simulink model "QuadArchitecture_AI"  (R2026b)
settings: Solver=VariableStepAuto
settings Model: DataDictionary=QuadInterfaces_AI.sldd  Creator=JonathanTee  LastModifiedBy=JonathanTee

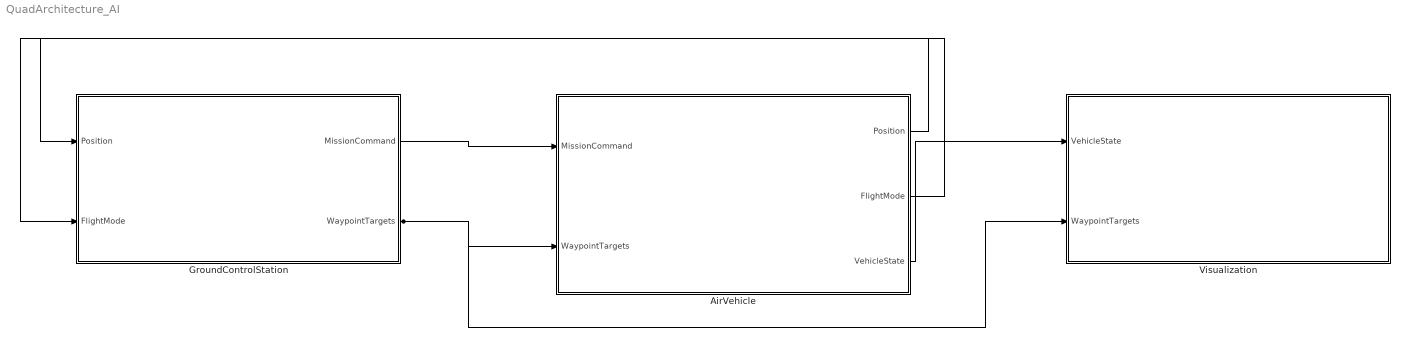
== system QuadArchitecture_AI ==
  AirVehicle : Subsystem
      settings: PortSchema="{\"entries\":[{\"content\":{\"headerSize\":26,\"margin\":15,\"minimumSpacing\":25,\"sides\":[{\"content\":{\"connectorIds\":[\"In1\",\"In2\"]},\"type\":\"ConnectorPlacement.EquallySpacedRectSide\",\"uuid\":\"ecfb2a5d-ebc3-4605-9a84-c6fd342510eb\"},{\"content\":{\"connectorIds\":[\"Out1\",\"Out2\",\"Out3\"],\"side\":\"RIGHT\"},\"type\":\"ConnectorPlacement.EquallySpacedRectSide\",\"uuid\":\"41ea779c-ccae-40c9-bf4c-62eb2a12d4ec\"},{\"content\":{\"side\":\"TOP\"},\"type\":\"ConnectorPlacement.EquallySpacedRectSide\",\"uuid\":\"f1fc56fa-babc-4d23-97d2-f02afcdd55d8\"}]},\"type\":\"ConnectorPlacement.EquallySpacedConnector\",\"uuid\":\"2007e49f-3d37-456e-85ff-e7f0d83353ae\"}],\"packageUris\":[\"http://schema.mathworks.com/mf0/Connector/R2020b\"],\"version\":\"1.0\"}"
  GroundControlStation : Subsystem
      settings: PortSchema="{\"entries\":[{\"content\":{\"headerSize\":26,\"margin\":15,\"minimumSpacing\":25,\"sides\":[{\"content\":{\"connectorIds\":[\"In1\",\"In2\"]},\"type\":\"ConnectorPlacement.EquallySpacedRectSide\",\"uuid\":\"ecfb2a5d-ebc3-4605-9a84-c6fd342510eb\"},{\"content\":{\"connectorIds\":[\"Out1\",\"Out2\"],\"side\":\"RIGHT\"},\"type\":\"ConnectorPlacement.EquallySpacedRectSide\",\"uuid\":\"41ea779c-ccae-40c9-bf4c-62eb2a12d4ec\"},{\"content\":{\"side\":\"TOP\"},\"type\":\"ConnectorPlacement.EquallySpacedRectSide\",\"uuid\":\"f1fc56fa-babc-4d23-97d2-f02afcdd55d8\"}]},\"type\":\"ConnectorPlacement.EquallySpacedConnector\",\"uuid\":\"2007e49f-3d37-456e-85ff-e7f0d83353ae\"}],\"packageUris\":[\"http://schema.mathworks.com/mf0/Connector/R2020b\"],\"version\":\"1.0\"}"
  Visualization : Subsystem
      settings: PortSchema="{\"entries\":[{\"content\":{\"headerSize\":26,\"margin\":15,\"minimumSpacing\":25,\"sides\":[{\"content\":{\"connectorIds\":[\"In1\",\"In2\"]},\"type\":\"ConnectorPlacement.EquallySpacedRectSide\",\"uuid\":\"ecfb2a5d-ebc3-4605-9a84-c6fd342510eb\"},{\"content\":{\"side\":\"RIGHT\"},\"type\":\"ConnectorPlacement.EquallySpacedRectSide\",\"uuid\":\"41ea779c-ccae-40c9-bf4c-62eb2a12d4ec\"},{\"content\":{\"side\":\"TOP\"},\"type\":\"ConnectorPlacement.EquallySpacedRectSide\",\"uuid\":\"f1fc56fa-babc-4d23-97d2-f02afcdd55d8\"}]},\"type\":\"ConnectorPlacement.EquallySpacedConnector\",\"uuid\":\"2007e49f-3d37-456e-85ff-e7f0d83353ae\"}],\"packageUris\":[\"http://schema.mathworks.com/mf0/Connector/R2020b\"],\"version\":\"1.0\"}"
  wires:
  AirVehicle/3(VehicleState) -> Visualization/1(VehicleState)
  AirVehicle/2(FlightMode) -> GroundControlStation/2(FlightMode)
  AirVehicle/1(Position) -> GroundControlStation/1(Position)
  GroundControlStation/2(WaypointTargets) -> Visualization/2(WaypointTargets), AirVehicle/2(WaypointTargets)
  GroundControlStation/1(MissionCommand) -> AirVehicle/1(MissionCommand)

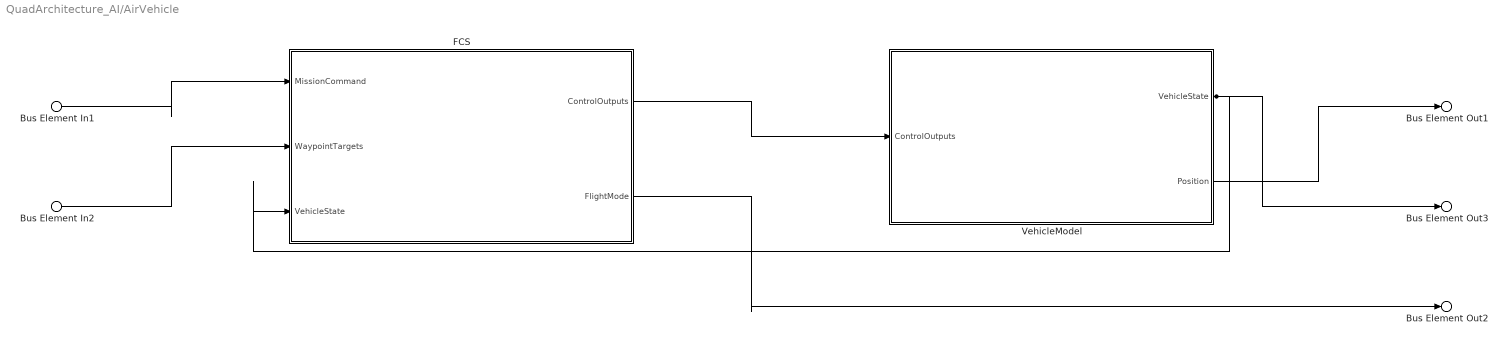
== system QuadArchitecture_AI/AirVehicle ==
  Bus Element In1 : Inport  PortName=MissionCommand
  Bus Element In2 : Inport  Port=2  PortName=WaypointTargets
  FCS : Subsystem
      settings: PortSchema="{\"entries\":[{\"content\":{\"headerSize\":26,\"margin\":15,\"minimumSpacing\":25,\"sides\":[{\"content\":{\"connectorIds\":[\"In1\",\"In2\",\"In3\"]},\"type\":\"ConnectorPlacement.EquallySpacedRectSide\",\"uuid\":\"ecfb2a5d-ebc3-4605-9a84-c6fd342510eb\"},{\"content\":{\"connectorIds\":[\"Out1\",\"Out2\"],\"side\":\"RIGHT\"},\"type\":\"ConnectorPlacement.EquallySpacedRectSide\",\"uuid\":\"41ea779c-ccae-40c9-bf4c-62eb2a12d4ec\"},{\"content\":{\"side\":\"TOP\"},\"type\":\"ConnectorPlacement.EquallySpacedRectSide\",\"uuid\":\"f1fc56fa-babc-4d23-97d2-f02afcdd55d8\"}]},\"type\":\"ConnectorPlacement.EquallySpacedConnector\",\"uuid\":\"2007e49f-3d37-456e-85ff-e7f0d83353ae\"}],\"packageUris\":[\"http://schema.mathworks.com/mf0/Connector/R2020b\"],\"version\":\"1.0\"}"
  VehicleModel : Subsystem
      settings: PortSchema="{\"entries\":[{\"content\":{\"headerSize\":26,\"margin\":15,\"minimumSpacing\":25,\"sides\":[{\"content\":{\"connectorIds\":[\"In1\"]},\"type\":\"ConnectorPlacement.EquallySpacedRectSide\",\"uuid\":\"ecfb2a5d-ebc3-4605-9a84-c6fd342510eb\"},{\"content\":{\"connectorIds\":[\"Out1\",\"Out2\"],\"side\":\"RIGHT\"},\"type\":\"ConnectorPlacement.EquallySpacedRectSide\",\"uuid\":\"41ea779c-ccae-40c9-bf4c-62eb2a12d4ec\"},{\"content\":{\"side\":\"TOP\"},\"type\":\"ConnectorPlacement.EquallySpacedRectSide\",\"uuid\":\"f1fc56fa-babc-4d23-97d2-f02afcdd55d8\"}]},\"type\":\"ConnectorPlacement.EquallySpacedConnector\",\"uuid\":\"2007e49f-3d37-456e-85ff-e7f0d83353ae\"}],\"packageUris\":[\"http://schema.mathworks.com/mf0/Connector/R2020b\"],\"version\":\"1.0\"}"
  Bus Element Out1 : Outport  PortName=Position
  Bus Element Out2 : Outport  Port=2  PortName=FlightMode
  Bus Element Out3 : Outport  Port=3  PortName=VehicleState
  wires:
  FCS/2(FlightMode) -> Bus Element Out2/1
  VehicleModel/2(Position) -> Bus Element Out1/1
  VehicleModel/1(VehicleState) -> Bus Element Out3/1, FCS/3(VehicleState)
  FCS/1(ControlOutputs) -> VehicleModel/1(ControlOutputs)
  Bus Element In2/1 -> FCS/2(WaypointTargets)
  Bus Element In1/1 -> FCS/1(MissionCommand)

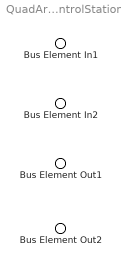
== system QuadArchitecture_AI/GroundControlStation ==
  Bus Element In1 : Inport  PortName=Position
  Bus Element In2 : Inport  Port=2  PortName=FlightMode
  Bus Element Out1 : Outport  PortName=MissionCommand
  Bus Element Out2 : Outport  Port=2  PortName=WaypointTargets

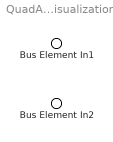
== system QuadArchitecture_AI/Visualization ==
  Bus Element In1 : Inport  PortName=VehicleState
  Bus Element In2 : Inport  Port=2  PortName=WaypointTargets

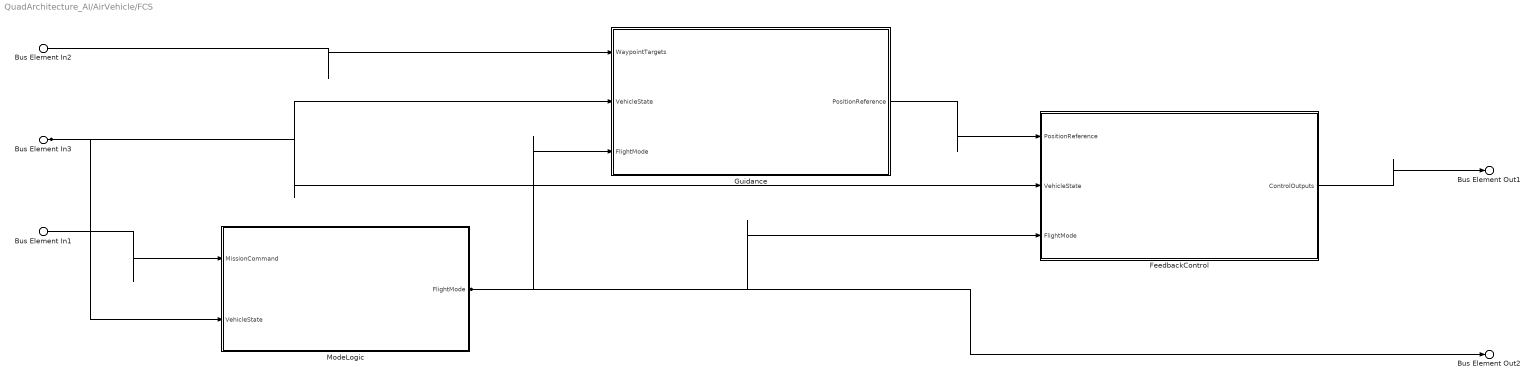
== system QuadArchitecture_AI/AirVehicle/FCS ==
  Bus Element In1 : Inport  PortName=MissionCommand
  Bus Element In2 : Inport  Port=2  PortName=WaypointTargets
  Bus Element In3 : Inport  Port=3  PortName=VehicleState
  FeedbackControl : Subsystem
      settings: PortSchema="{\"entries\":[{\"content\":{\"headerSize\":26,\"margin\":15,\"minimumSpacing\":25,\"sides\":[{\"content\":{\"connectorIds\":[\"In1\",\"In2\",\"In3\"]},\"type\":\"ConnectorPlacement.EquallySpacedRectSide\",\"uuid\":\"ecfb2a5d-ebc3-4605-9a84-c6fd342510eb\"},{\"content\":{\"connectorIds\":[\"Out1\"],\"side\":\"RIGHT\"},\"type\":\"ConnectorPlacement.EquallySpacedRectSide\",\"uuid\":\"41ea779c-ccae-40c9-bf4c-62eb2a12d4ec\"},{\"content\":{\"side\":\"TOP\"},\"type\":\"ConnectorPlacement.EquallySpacedRectSide\",\"uuid\":\"f1fc56fa-babc-4d23-97d2-f02afcdd55d8\"}]},\"type\":\"ConnectorPlacement.EquallySpacedConnector\",\"uuid\":\"2007e49f-3d37-456e-85ff-e7f0d83353ae\"}],\"packageUris\":[\"http://schema.mathworks.com/mf0/Connector/R2020b\"],\"version\":\"1.0\"}"
  Guidance : Subsystem
      settings: PortSchema="{\"entries\":[{\"content\":{\"headerSize\":26,\"margin\":15,\"minimumSpacing\":25,\"sides\":[{\"content\":{\"connectorIds\":[\"In1\",\"In2\",\"In3\"]},\"type\":\"ConnectorPlacement.EquallySpacedRectSide\",\"uuid\":\"ecfb2a5d-ebc3-4605-9a84-c6fd342510eb\"},{\"content\":{\"connectorIds\":[\"Out1\"],\"side\":\"RIGHT\"},\"type\":\"ConnectorPlacement.EquallySpacedRectSide\",\"uuid\":\"41ea779c-ccae-40c9-bf4c-62eb2a12d4ec\"},{\"content\":{\"side\":\"TOP\"},\"type\":\"ConnectorPlacement.EquallySpacedRectSide\",\"uuid\":\"f1fc56fa-babc-4d23-97d2-f02afcdd55d8\"}]},\"type\":\"ConnectorPlacement.EquallySpacedConnector\",\"uuid\":\"2007e49f-3d37-456e-85ff-e7f0d83353ae\"}],\"packageUris\":[\"http://schema.mathworks.com/mf0/Connector/R2020b\"],\"version\":\"1.0\"}"
  ModeLogic : Subsystem
      settings: PortSchema="{\"entries\":[{\"content\":{\"headerSize\":26,\"margin\":15,\"minimumSpacing\":25,\"sides\":[{\"content\":{\"connectorIds\":[\"In1\",\"In2\"]},\"type\":\"ConnectorPlacement.EquallySpacedRectSide\",\"uuid\":\"ecfb2a5d-ebc3-4605-9a84-c6fd342510eb\"},{\"content\":{\"connectorIds\":[\"Out1\"],\"side\":\"RIGHT\"},\"type\":\"ConnectorPlacement.EquallySpacedRectSide\",\"uuid\":\"41ea779c-ccae-40c9-bf4c-62eb2a12d4ec\"},{\"content\":{\"side\":\"TOP\"},\"type\":\"ConnectorPlacement.EquallySpacedRectSide\",\"uuid\":\"f1fc56fa-babc-4d23-97d2-f02afcdd55d8\"}]},\"type\":\"ConnectorPlacement.EquallySpacedConnector\",\"uuid\":\"2007e49f-3d37-456e-85ff-e7f0d83353ae\"}],\"packageUris\":[\"http://schema.mathworks.com/mf0/Connector/R2020b\"],\"version\":\"1.0\"}"
  Bus Element Out1 : Outport  PortName=ControlOutputs
  Bus Element Out2 : Outport  Port=2  PortName=FlightMode
  wires:
  FeedbackControl/1(ControlOutputs) -> Bus Element Out1/1
  Guidance/1(PositionReference) -> FeedbackControl/1(PositionReference)
  ModeLogic/1(FlightMode) -> Bus Element Out2/1, FeedbackControl/3(FlightMode), Guidance/3(FlightMode)
  Bus Element In3/1 -> FeedbackControl/2(VehicleState), Guidance/2(VehicleState), ModeLogic/2(VehicleState)
  Bus Element In2/1 -> Guidance/1(WaypointTargets)
  Bus Element In1/1 -> ModeLogic/1(MissionCommand)

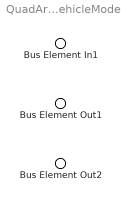
== system QuadArchitecture_AI/AirVehicle/VehicleModel ==
  Bus Element In1 : Inport  PortName=ControlOutputs
  Bus Element Out1 : Outport  PortName=VehicleState
  Bus Element Out2 : Outport  Port=2  PortName=Position

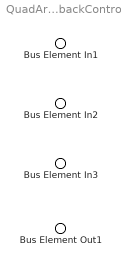
== system QuadArchitecture_AI/AirVehicle/FCS/FeedbackControl ==
  Bus Element In1 : Inport  PortName=PositionReference
  Bus Element In2 : Inport  Port=2  PortName=VehicleState
  Bus Element In3 : Inport  Port=3  PortName=FlightMode
  Bus Element Out1 : Outport  PortName=ControlOutputs

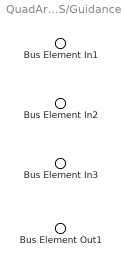
== system QuadArchitecture_AI/AirVehicle/FCS/Guidance ==
  Bus Element In1 : Inport  PortName=WaypointTargets
  Bus Element In2 : Inport  Port=2  PortName=VehicleState
  Bus Element In3 : Inport  Port=3  PortName=FlightMode
  Bus Element Out1 : Outport  PortName=PositionReference

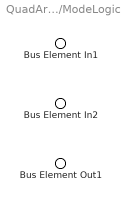
== system QuadArchitecture_AI/AirVehicle/FCS/ModeLogic ==
  Bus Element In1 : Inport  PortName=MissionCommand
  Bus Element In2 : Inport  Port=2  PortName=VehicleState
  Bus Element Out1 : Outport  PortName=FlightMode
